simulink model "L2_scheme"  (R2023b)
settings: Solver=VariableStepAuto  StartTime=0.0  StopTime=10.0  RelTol=1e-3
libraries: dspsrcs4 x1
settings Model: Creator=vladi  LastModifiedBy=vladi

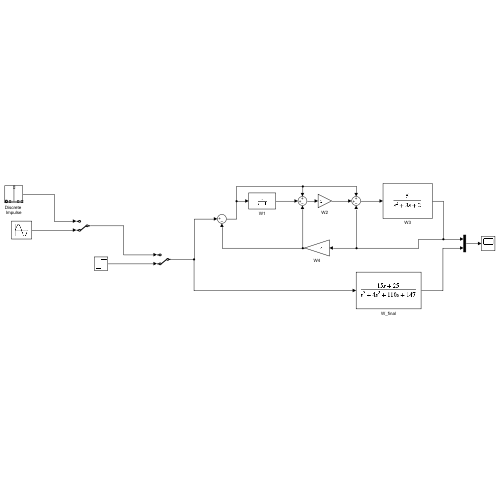
[thumbnail: Simulink's stored preview of the top-level diagram]
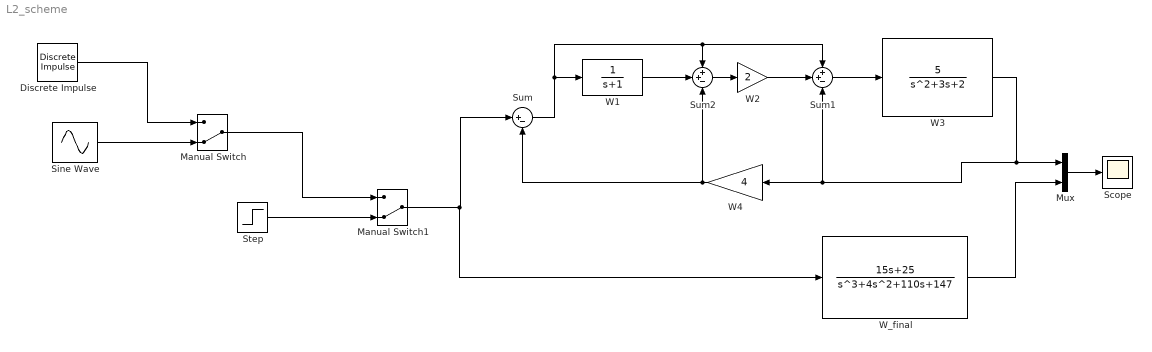
== system L2_scheme ==
  Discrete Impulse : dspsrcs4/Discrete  Impulse  Delay=0  SampleTime=1  FrameSample=1  OutputFrames=off  dataType=double  isSigned=on  wordLen=16  udDataType=sfix(16)  fracBitsMode=Best precision  numFracBits=15  OutDataTypeStr=double  LastOutDataTypeStr=double
  Manual Switch : ManualSwitch  CurrentSetting=0
  Manual Switch1 : ManualSwitch  CurrentSetting=0
  Mux : Mux  Inputs=2
  Scope : Scope
  Sine Wave : Sin  SampleTime=0
  Step : Step  SampleTime=0
  Sum : Sum  Inputs=|+-
  Sum1 : Sum  Inputs=++-
  Sum2 : Sum  Inputs=++-
  W1 : TransferFcn  Denominator=[1 1]
  W2 : Gain  Gain=2
  W3 : TransferFcn  Numerator=[5]  Denominator=[1 3 2]
  W4 : Gain  Gain=4
  W_final : TransferFcn  Numerator=[15 25]  Denominator=[1 4 110 147]
  wires:
  Sum/1 -> Sum2/1, Sum1/1, W1/1
  Sum2/1 -> W2/1
  W2/1 -> Sum1/2
  Sum1/1 -> W3/1
  W1/1 -> Sum2/2
  W4/1 -> Sum/2, Sum2/3
  W3/1 -> Sum1/3, W4/1, Mux/1
  Mux/1 -> Scope/1
  W_final/1 -> Mux/2
  Discrete Impulse/1 -> Manual Switch/1
  Sine Wave/1 -> Manual Switch/2
  Manual Switch1/1 -> W_final/1, Sum/1
  Step/1 -> Manual Switch1/2
  Manual Switch/1 -> Manual Switch1/1
